simulink model "Sistema_Control_01"  (R2026a)
settings: Solver=VariableStepAuto
settings Model: Creator=Lorenzo  LastModifiedBy=Lorenzo

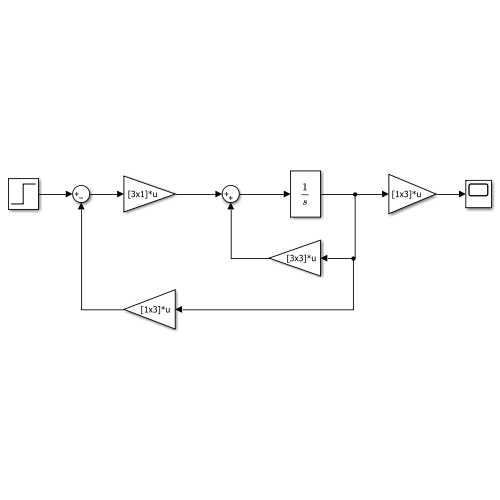
[thumbnail: Simulink's stored preview of the top-level diagram]
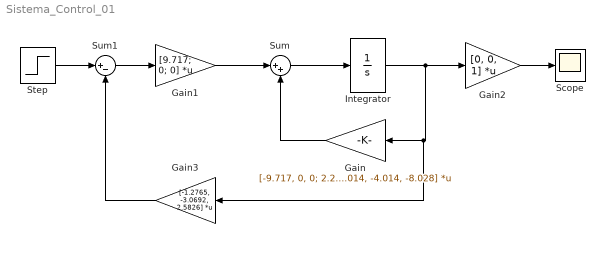
== system Sistema_Control_01 ==
  Gain : Gain  Gain=[-9.717, 0, 0; 2.209, -6.658, -2.209; 4.014, -4.014, -8.028]  Multiplication=Matrix(K*u)
  Gain1 : Gain  Gain=[9.717; 0; 0]  Multiplication=Matrix(K*u)
  Gain2 : Gain  Gain=[0, 0, 1]  Multiplication=Matrix(K*u)
  Gain3 : Gain  Gain=[-1.2765, -3.0692, 2.5826]  Multiplication=Matrix(K*u)
  Integrator : Integrator
  Scope : Scope
      settings: ActiveDisplayYMinimum=-3.3933862211836865  ActiveDisplayYMaximum=4.8388849695794942
  Step : Step  SampleTime=0
  Sum : Sum  Inputs=|++
  Sum1 : Sum  Inputs=|+-
  wires:
  Step/1 -> Sum1/1
  Sum1/1 -> Gain1/1
  Sum/1 -> Integrator/1
  Integrator/1 -> Gain3/1, Gain/1, Gain2/1
  Gain2/1 -> Scope/1
  Gain/1 -> Sum/2
  Gain3/1 -> Sum1/2
  Gain1/1 -> Sum/1
